simulink subsystem "wmech_Calc"  (R2025b)
settings: Solver=VariableStepAuto
undefined symbols (not defined in the file): FCS
settings Model: Creator=kara  LastModifiedBy=Cheng
settings RTWCC: GPUComputeCapability=3.5

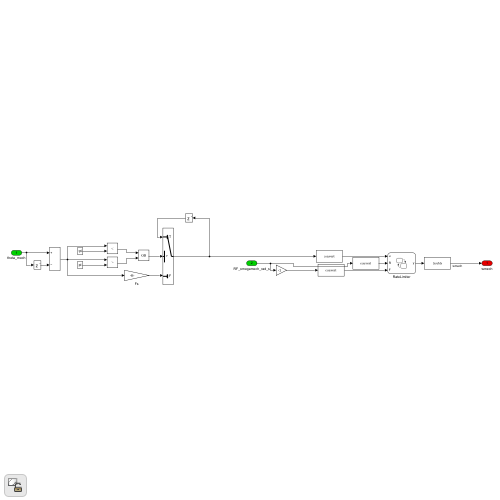
[thumbnail: Simulink's stored preview of the top-level diagram]
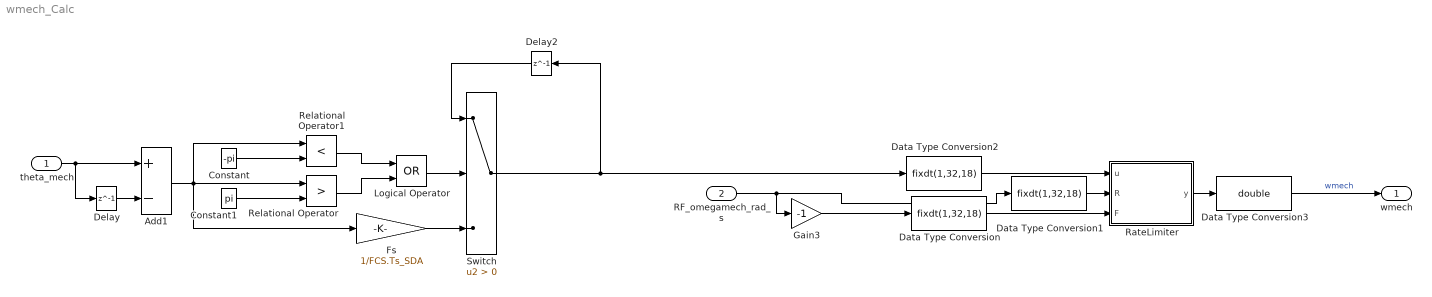
== system wmech_Calc ==
  theta_mech : Inport
  RF_omegamech_rad_s : Inport  Port=2
  Add1 : Sum  Inputs=+-  OutDataTypeStr=HighScaling  SaturateOnIntegerOverflow=on
  Constant : Constant  Value=-pi  OutDataTypeStr=HighScaling
  Constant1 : Constant  Value=pi  OutDataTypeStr=HighScaling
  Data Type Conversion : DataTypeConversion  OutDataTypeStr=fixdt(1,32,18)  SaturateOnIntegerOverflow=off  RndMeth=Floor
  Data Type Conversion1 : DataTypeConversion  OutDataTypeStr=fixdt(1,32,18)  SaturateOnIntegerOverflow=off  RndMeth=Floor
  Data Type Conversion2 : DataTypeConversion  OutDataTypeStr=fixdt(1,32,18)  SaturateOnIntegerOverflow=off  RndMeth=Floor
  Data Type Conversion3 : DataTypeConversion  OutDataTypeStr=double  SaturateOnIntegerOverflow=off  RndMeth=Floor
  Delay : Delay  DelayLength=1
  Delay2 : Delay  DelayLength=1
  Fs : Gain  Gain=1/FCS.Ts_SDA  OutDataTypeStr=SIScaling
  Gain3 : Gain  Gain=-1  OutDataTypeStr=SIScaling
  Logical Operator : Logic  Operator=OR  AllPortsSameDT=off  OutDataTypeStr=boolean
  RateLimiter : Stateflow chart  TreatAsAtomicUnit=on
  Relational Operator : RelationalOperator  Operator=>  OutDataTypeStr=boolean  RndMeth=Simplest  InputSameDT=off
  Relational Operator1 : RelationalOperator  Operator=<  OutDataTypeStr=boolean  RndMeth=Simplest  InputSameDT=off
  Switch : Switch  Criteria=u2 > Threshold  OutDataTypeStr=SIScaling  SaturateOnIntegerOverflow=off  InputSameDT=off
  wmech : Outport
  wires:
  theta_mech/1 -> Add1/1, Delay/1
  Delay/1 -> Add1/2
  Add1/1 -> Relational Operator/1, Relational Operator1/1, Fs/1
  Constant/1 -> Relational Operator1/2
  Constant1/1 -> Relational Operator/2
  Relational Operator1/1 -> Logical Operator/1
  Relational Operator/1 -> Logical Operator/2
  Fs/1 -> Switch/3
  Delay2/1 -> Switch/1
  Logical Operator/1 -> Switch/2
  Switch/1 -> Delay2/1, Data Type Conversion2/1
  Data Type Conversion2/1 -> RateLimiter/1(u)
  RF_omegamech_rad_s/1 -> Gain3/1, Data Type Conversion1/1
  Data Type Conversion1/1 -> RateLimiter/2(R)
  Gain3/1 -> Data Type Conversion/1
  Data Type Conversion/1 -> RateLimiter/3(F)
  Data Type Conversion3/1 -> wmech/1  "wmech"
  RateLimiter/1(y) -> Data Type Conversion3/1

== stateflow chart wmech_Calc/RateLimiter ==
  settings: updateMethod=DISCRETE  sampleTime=FCS.Ts_SDA
  state IDLE
  state Rising
    entry:  y =  fi(y_prev +dT * R, 1, 32, 18);
    exit: y_prev = y;
  state Falling
    entry:  y = fi(y_prev+dT * F, 1, 32, 18);
    exit: y_prev = y;
  state Directpassage
    entry:  y = u;
    exit: y_prev = y;
  (default) -> IDLE
  IDLE -> (junction 22)
  (junction 22) -> Rising [order 1] : [(u-y_prev)/dT>=R]
  (junction 22) -> Falling [order 2] : [(u-y_prev)/dT<=F]
  Rising -> (junction 22)
  Falling -> (junction 22)
  Directpassage -> (junction 22)
  (junction 22) -> Directpassage [order 3] : [(u-y_prev)/dT<R && (u-y_prev)/dT>F]
  data: u input fixdt(1,32,18); R input fixdt(1,32,18); F input fixdt(1,32,18); dT constant fixdt(1,32,18) size=1 =FOC.SampleTime.TsCur; y output fixdt(1,32,18); y_prev local fixdt(1,32,18) =0
